simulink model "v3_2025_10_25_D1_final"  (R2025a)
settings: Solver=FixedStepAuto  StartTime=0.0  StopTime=10.0  FixedStep=1e-3  RelTol=1e-3  EnableMultiTasking=on
undefined symbols (not defined in the file): D0, D1, D10, D11, D12, D13, D2, D3, D4, D5, D6, D7, D8, D9, PTA0, PTA1, PTA2, PTB23, PTB9, PTC16, PTC17, PTC2, PTC3, PTC4, PTD0, PTD1, PTD2, PTD3
libraries: frdmk64flib x14
settings Model: ExtModeTrigDuration=5  Creator=School Account  LastModifiedBy=School Account
settings OptimizationCC: DefaultParameterBehavior=Inlined  EnhancedBackFolding=on  PassReuseOutputArgsAs=Individual arguments  ZeroExternalMemoryAtStartup=off  ZeroInternalMemoryAtStartup=off  MaxStackSize=64  OptimizeBlockOrder=speed  DifferentSizesBufferReuse=on  OptimizationCustomize=off  EfficientTunableParamExpr=on
settings DebuggingCC: ParameterTunabilityLossMsg=error
settings HardwareCC: ProdBitPerPointer=32.0  ProdBitPerSizeT=32.0  ProdBitPerPtrDiffT=32.0  ProdLargestAtomicInteger=Long  ProdLargestAtomicFloat=Double  ProdWordSize=32.0  ProdHWDeviceType=ARM Compatible->ARM Cortex
settings SFSimCC: MATLABDynamicMemAlloc=off
settings RTWCC: SystemTargetFile=ert.tlc  HardwareBoard=NXP FRDM-K64F  TLCOptions="-aInlineSetEventsForThisBaseRateFcn=TLC_FALSE -aSuppressMultiTaskScheduler=TLC_FALSE  -aRateBasedStepFcn=0"  TemplateMakefile=ert_default_tmf  Toolchain=GNU Tools for ARM Embedded Processors  Description=Embedded Coder
settings CodeAppCC: ForceParamTrailComments=on  IgnoreCustomStorageClasses=off  OperatorAnnotations=on  SimulinkDataObjDesc=on  SFDataObjDesc=on  InsertBlockDesc=on
settings ERTTargetCC: ExtModeTransport=4.0  ExtModeStaticAlloc=off  ExtModeMexFile=sendToCommService  ExtModeIntrfLevel=Level1

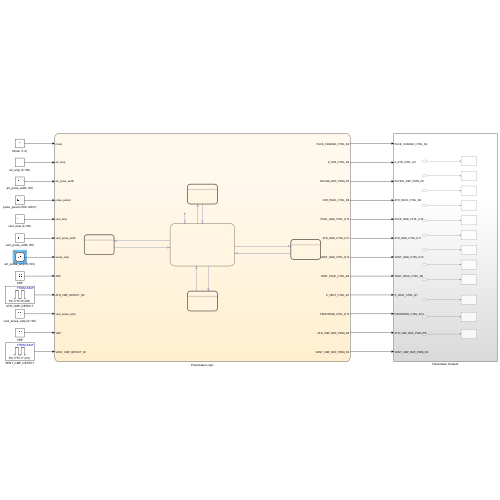
[thumbnail: Simulink's stored preview of the top-level diagram]
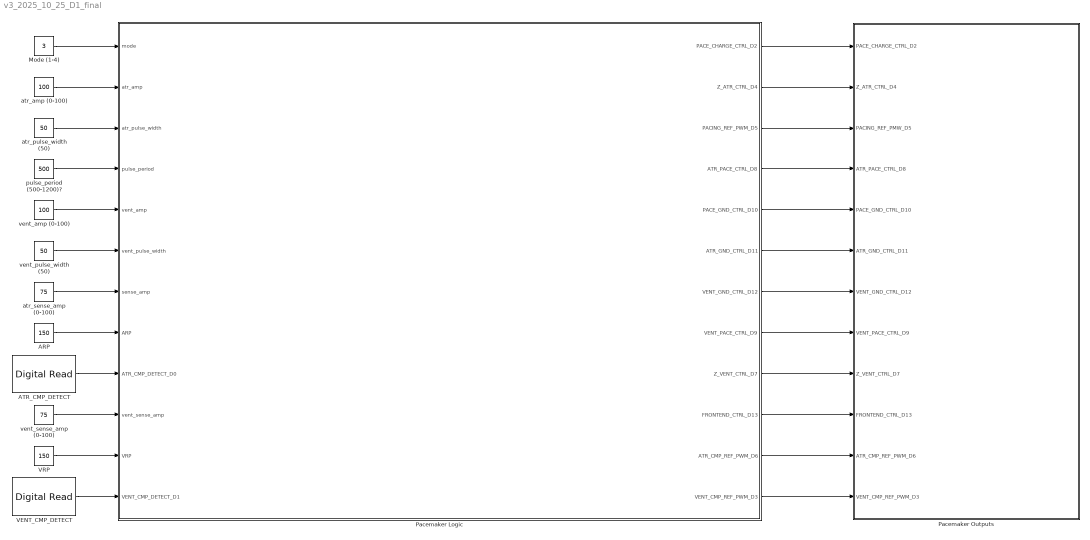
== system v3_2025_10_25_D1_final ==
  ARP : Constant  Value=150
  ATR_CMP_DETECT : frdmk64flib/Digital Read  Whichpin=PTC16 (D0)  SampleTime=-1
  Mode (1-4) : Constant  Value=3
  Pacemaker Logic : Stateflow chart  TreatAsAtomicUnit=on
  Pacemaker Outputs : Subsystem
  VENT_CMP_DETECT : frdmk64flib/Digital Read  Whichpin=PTC17 (D1)  SampleTime=-1
  VRP : Constant  Value=150
  atr_amp (0-100) : Constant  Value=100
  atr_pulse_width (50) : Constant  Value=50
  atr_sense_amp (0-100) : Constant  Value=75
  pulse_period (500-1200)? : Constant  Value=500
  vent_amp (0-100) : Constant  Value=100
  vent_pulse_width (50) : Constant  Value=50
  vent_sense_amp (0-100) : Constant  Value=75
  wires:
  Mode (1-4)/1 -> Pacemaker Logic/1(mode)
  atr_amp (0-100)/1 -> Pacemaker Logic/2(atr_amp)
  atr_pulse_width (50)/1 -> Pacemaker Logic/3(atr_pulse_width)
  pulse_period (500-1200)?/1 -> Pacemaker Logic/4(pulse_period)
  Pacemaker Logic/1(PACE_CHARGE_CTRL_D2) -> Pacemaker Outputs/1(PACE_CHARGE_CTRL_D2)
  Pacemaker Logic/2(Z_ATR_CTRL_D4) -> Pacemaker Outputs/2(Z_ATR_CTRL_D4)
  Pacemaker Logic/3(PACING_REF_PWM_D5) -> Pacemaker Outputs/3(PACING_REF_PMW_D5)
  Pacemaker Logic/4(ATR_PACE_CTRL_D8) -> Pacemaker Outputs/4(ATR_PACE_CTRL_D8)
  Pacemaker Logic/5(PACE_GND_CTRL_D10) -> Pacemaker Outputs/5(PACE_GND_CTRL_D10)
  Pacemaker Logic/6(ATR_GND_CTRL_D11) -> Pacemaker Outputs/6(ATR_GND_CTRL_D11)
  vent_amp (0-100)/1 -> Pacemaker Logic/5(vent_amp)
  vent_pulse_width (50)/1 -> Pacemaker Logic/6(vent_pulse_width)
  Pacemaker Logic/7(VENT_GND_CTRL_D12) -> Pacemaker Outputs/7(VENT_GND_CTRL_D12)
  Pacemaker Logic/8(VENT_PACE_CTRL_D9) -> Pacemaker Outputs/8(VENT_PACE_CTRL_D9)
  Pacemaker Logic/9(Z_VENT_CTRL_D7) -> Pacemaker Outputs/9(Z_VENT_CTRL_D7)
  atr_sense_amp (0-100)/1 -> Pacemaker Logic/7(sense_amp)
  ARP/1 -> Pacemaker Logic/8(ARP)
  ATR_CMP_DETECT/1 -> Pacemaker Logic/9(ATR_CMP_DETECT_D0)
  Pacemaker Logic/10(FRONTEND_CTRL_D13) -> Pacemaker Outputs/10(FRONTEND_CTRL_D13)
  Pacemaker Logic/11(ATR_CMP_REF_PWM_D6) -> Pacemaker Outputs/11(ATR_CMP_REF_PWM_D6)
  Pacemaker Logic/12(VENT_CMP_REF_PWM_D3) -> Pacemaker Outputs/12(VENT_CMP_REF_PWM_D3)
  vent_sense_amp (0-100)/1 -> Pacemaker Logic/10(vent_sense_amp)
  VRP/1 -> Pacemaker Logic/11(VRP)
  VENT_CMP_DETECT/1 -> Pacemaker Logic/12(VENT_CMP_DETECT_D1)

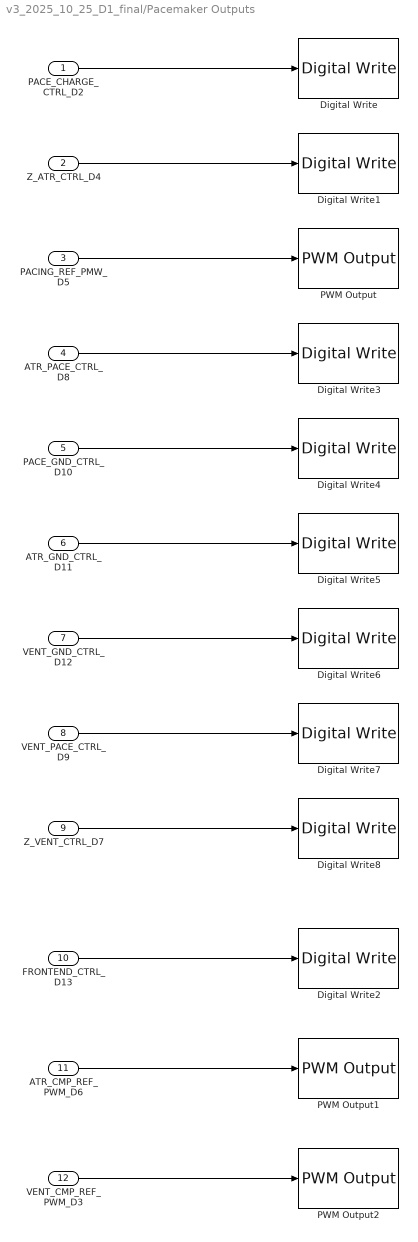
== system v3_2025_10_25_D1_final/Pacemaker Outputs ==
  PACE_CHARGE_CTRL_D2 : Inport
  Z_ATR_CTRL_D4 : Inport  Port=2
  PACING_REF_PMW_D5 : Inport  Port=3
  ATR_PACE_CTRL_D8 : Inport  Port=4
  PACE_GND_CTRL_D10 : Inport  Port=5
  ATR_GND_CTRL_D11 : Inport  Port=6
  VENT_GND_CTRL_D12 : Inport  Port=7
  VENT_PACE_CTRL_D9 : Inport  Port=8
  Z_VENT_CTRL_D7 : Inport  Port=9
  FRONTEND_CTRL_D13 : Inport  Port=10
  ATR_CMP_REF_PWM_D6 : Inport  Port=11
  VENT_CMP_REF_PWM_D3 : Inport  Port=12
  Digital Write : frdmk64flib/Digital Write  Whichpin=PTB9 (D2)
  Digital Write1 : frdmk64flib/Digital Write  Whichpin=PTB23 (D4)
  Digital Write2 : frdmk64flib/Digital Write  Whichpin=PTD1 (D13)
  Digital Write3 : frdmk64flib/Digital Write  Whichpin=PTA0 (D8)
  Digital Write4 : frdmk64flib/Digital Write  Whichpin=PTD0 (D10)
  Digital Write5 : frdmk64flib/Digital Write  Whichpin=PTD2 (D11)
  Digital Write6 : frdmk64flib/Digital Write  Whichpin=PTD3 (D12)
  Digital Write7 : frdmk64flib/Digital Write  Whichpin=PTC4 (D9)
  Digital Write8 : frdmk64flib/Digital Write  Whichpin=PTC3 (D7)
  PWM Output : frdmk64flib/PWM Output  Whichpin=PTA2 (D5)  InitialFrequency=2000  InitialDutyCycle=0
  PWM Output1 : frdmk64flib/PWM Output  Whichpin=PTC2 (D6)  InitialFrequency=2000  InitialDutyCycle=0
  PWM Output2 : frdmk64flib/PWM Output  Whichpin=PTA1 (D3)  InitialFrequency=2000  InitialDutyCycle=0
  wires:
  PACE_CHARGE_CTRL_D2/1 -> Digital Write/1
  Z_ATR_CTRL_D4/1 -> Digital Write1/1
  PACING_REF_PMW_D5/1 -> PWM Output/1
  ATR_PACE_CTRL_D8/1 -> Digital Write3/1
  PACE_GND_CTRL_D10/1 -> Digital Write4/1
  ATR_GND_CTRL_D11/1 -> Digital Write5/1
  VENT_GND_CTRL_D12/1 -> Digital Write6/1
  VENT_PACE_CTRL_D9/1 -> Digital Write7/1
  Z_VENT_CTRL_D7/1 -> Digital Write8/1
  FRONTEND_CTRL_D13/1 -> Digital Write2/1
  ATR_CMP_REF_PWM_D6/1 -> PWM Output1/1
  VENT_CMP_REF_PWM_D3/1 -> PWM Output2/1

== stateflow chart v3_2025_10_25_D1_final/Pacemaker Logic ==
  state AAI
    state AAI_Charge
      entry:
      FRONTEND_CTRL_D13 = 1;
      %Charging C22
      ATR_PACE_CTRL_D8 = 0;
      VENT_PACE_CTRL_D9 = 0;
      PACING_REF_PWM_D5 = atr_amp;
      PACE_CHARGE_CTRL_D2 = 1;
      %Discharging C21
      PACE_GND_CTRL_D10 = 1;
      ATR_PACE_CTRL_D8 = 0;
      Z_VENT_CTRL_D7 = 0;
      Z_ATR_CTRL_D4 = 0;
      VENT_PACE_CTRL_D9 = 0;
      VENT_GND_CTRL_D12 = 0;
      ATR_GND_CTRL_D11 = 1;
      ATR_CMP_REF_PWM_D6 = sense_amp;
    state AAI_Pace
      entry:
      %Pacing
      PACE_CHARGE_CTRL_D2 = 0;
      PACE_GND_CTRL_D10= 1;
      VENT_PACE_CTRL_D9 = 0;
      VENT_GND_CTRL_D12= 0;
      Z_VENT_CTRL_D7 = 0;
      Z_ATR_CTRL_D4 = 0;
      ATR_GND_CTRL_D11 = 0;
      ATR_PACE_CTRL_D8 = 1;
    state AAI_Inhibit
      entry:
      FRONTEND_CTRL_D13 = 0;
      %Charging C22
      ATR_PACE_CTRL_D8 = 0;
      VENT_PACE_CTRL_D9 = 0;
      PACING_REF_PWM_D5 = atr_amp;
      PACE_CHARGE_CTRL_D2 = 1;
      %Discharging C21
      PACE_GND_CTRL_D10 = 1;
      ATR_PACE_CTRL_D8 = 0;
      Z_VENT_CTRL_D7 = 0;
      Z_ATR_CTRL_D4 = 0;
      VENT_PACE_CTRL_D9 = 0;
      VENT_GND_CTRL_D12 = 0;
      ATR_GND_CTRL_D11 = 1;
      ATR_CMP_REF_PWM_D6 = sense_amp;
    (default) -> AAI_Charge
    AAI_Charge -> AAI_Pace [order 1] : [after(pulse_period - atr_pulse_width - ARP,msec)]
    AAI_Pace -> AAI_Charge [order 1] : [after(atr_pulse_width,msec)]
    AAI_Charge -> (junction 58) [order 2] : [ATR_CMP_DETECT_D0 == 1]
    (junction 58) -> AAI_Inhibit : [after(atr_pulse_width,msec)]
    AAI_Pace -> AAI_Inhibit [order 2] : [after(atr_pulse_width,msec)]
    AAI_Inhibit -> AAI_Charge : [after(ARP, msec)]
  state Start
  state AOO
    state AOO_Charge
      entry:
      %Charging C22
      ATR_PACE_CTRL_D8 = 0;
      VENT_PACE_CTRL_D9 = 0;
      PACING_REF_PWM_D5 = atr_amp;
      PACE_CHARGE_CTRL_D2 = 1;
      %Discharging C21
      PACE_GND_CTRL_D10 = 1;
      ATR_PACE_CTRL_D8 = 0;
      Z_VENT_CTRL_D7 = 0;
      Z_ATR_CTRL_D4 = 0;
      VENT_PACE_CTRL_D9 = 0;
      VENT_GND_CTRL_D12 = 0;
      ATR_GND_CTRL_D11 = 1;
    state AOO_Pace
      entry:
      %Pacing
      PACE_CHARGE_CTRL_D2 = 0;
      PACE_GND_CTRL_D10= 1;
      VENT_PACE_CTRL_D9 = 0;
      VENT_GND_CTRL_D12= 0;
      Z_VENT_CTRL_D7 = 0;
      Z_ATR_CTRL_D4 = 0;
      ATR_GND_CTRL_D11 = 0;
      ATR_PACE_CTRL_D8 = 1;
    (default) -> AOO_Charge
    AOO_Charge -> AOO.AOO_Pace : [after(pulse_period - atr_pulse_width,msec)]
    AOO.AOO_Pace -> AOO_Charge : [after(atr_pulse_width,msec)]
  state VOO
    state VOO_Charge
      entry:
      %Charging C22
      VENT_PACE_CTRL_D9 = 0;
      ATR_PACE_CTRL_D8 = 0;
      PACING_REF_PWM_D5 = vent_amp;
      PACE_CHARGE_CTRL_D2 = 1;
      %Discharging C21
      PACE_GND_CTRL_D10 = 1;
      VENT_PACE_CTRL_D9 = 0;
      Z_ATR_CTRL_D4 = 0;
      Z_VENT_CTRL_D7 = 0;
      ATR_PACE_CTRL_D8 = 0;
      ATR_GND_CTRL_D11 = 0;
      VENT_GND_CTRL_D12 = 1;
    state AOO_Pace
      entry:
      %Pacing
      PACE_CHARGE_CTRL_D2 = 0;
      PACE_GND_CTRL_D10= 1;
      ATR_PACE_CTRL_D8 = 0;
      ATR_GND_CTRL_D11= 0;
      Z_ATR_CTRL_D4 = 0;
      Z_VENT_CTRL_D7 = 0;
      VENT_GND_CTRL_D12 = 0;
      VENT_PACE_CTRL_D9 = 1;
    (default) -> VOO_Charge
    VOO_Charge -> VOO.AOO_Pace : [after(pulse_period - vent_pulse_width,msec)]
    VOO.AOO_Pace -> VOO_Charge : [after(vent_pulse_width,msec)]
  state VVI
    state VVI_Charge
      entry:
      FRONTEND_CTRL_D13 = 1;
      %Charging C22
      VENT_PACE_CTRL_D9 = 0;
      ATR_PACE_CTRL_D8 = 0;
      PACING_REF_PWM_D5 = vent_amp;
      PACE_CHARGE_CTRL_D2 = 1;
      %Discharging C21
      PACE_GND_CTRL_D10 = 1;
      VENT_PACE_CTRL_D9 = 0;
      Z_ATR_CTRL_D4 = 0;
      Z_VENT_CTRL_D7 = 0;
      ATR_PACE_CTRL_D8 = 0;
      ATR_GND_CTRL_D11 = 0;
      VENT_GND_CTRL_D12 = 1;
      VENT_CMP_REF_PWM_D3 = vent_sense_amp;
    state VVI_Pace
      entry:
      %Pacing
      PACE_CHARGE_CTRL_D2 = 0;
      PACE_GND_CTRL_D10= 1;
      ATR_PACE_CTRL_D8 = 0;
      ATR_GND_CTRL_D11= 0;
      Z_ATR_CTRL_D4 = 0;
      Z_VENT_CTRL_D7 = 0;
      VENT_GND_CTRL_D12 = 0;
      VENT_PACE_CTRL_D9 = 1;
    state VVI_Inhibit
      entry:
      FRONTEND_CTRL_D13 = 0;
      %Charging C22
      VENT_PACE_CTRL_D9 = 0;
      ATR_PACE_CTRL_D8 = 0;
      PACING_REF_PWM_D5 = vent_amp;
      PACE_CHARGE_CTRL_D2 = 1;
      %Discharging C21
      PACE_GND_CTRL_D10 = 1;
      VENT_PACE_CTRL_D9 = 0;
      Z_VENT_CTRL_D7 = 0;
      Z_ATR_CTRL_D4 = 0;
      ATR_PACE_CTRL_D8 = 0;
      ATR_GND_CTRL_D11 = 0;
      VENT_GND_CTRL_D12 = 1;
      VENT_CMP_REF_PWM_D3 = vent_sense_amp;
    (default) -> VVI_Charge
    VVI_Charge -> VVI_Pace [order 1] : [after(pulse_period - vent_pulse_width - VRP,msec)]
    VVI_Pace -> VVI_Charge [order 1] : [after(vent_pulse_width,msec)]
    VVI_Charge -> (junction 65) [order 2] : [VENT_CMP_DETECT_D1 == 1]
    (junction 65) -> VVI_Inhibit : [after(vent_pulse_width,msec)]
    VVI_Pace -> VVI_Inhibit [order 2] : [after(vent_pulse_width,msec)]
    VVI_Inhibit -> VVI_Charge : [after(VRP, msec)]
  Start -> AAI [order 3] : [mode == 3]
  AAI -> Start : [mode ~= 3]
  (default) -> Start
  Start -> AOO [order 2] : [mode == 1]
  Start -> VOO [order 1] : [mode == 2]
  AOO -> Start : [mode ~= 1]
  VOO -> Start : [mode ~= 2]
  VVI -> Start : [mode ~= 4]
  Start -> VVI [order 4] : [mode == 4]
  data: PACE_CHARGE_CTRL_D2 output; Z_ATR_CTRL_D4 output; PACING_REF_PWM_D5 output; mode input; ATR_PACE_CTRL_D8 output; PACE_GND_CTRL_D10 output; atr_amp input; ATR_GND_CTRL_D11 output; atr_pulse_width input; pulse_period input; vent_amp input; VENT_GND_CTRL_D12 output; VENT_PACE_CTRL_D9 output; Z_VENT_CTRL_D7 output; vent_pulse_width input; FRONTEND_CTRL_D13 output; ATR_CMP_REF_PWM_D6 output; sense_amp input; ARP input; ATR_CMP_DETECT_D0 input; vent_sense_amp input; VENT_CMP_REF_PWM_D3 output; VRP input; VENT_CMP_DETECT_D1 input
